simulink model "IEEE_BUS_68_Baseline"  (R2025a)
settings: Solver=ode23tb  StartTime=0.0  StopTime=150  FixedStep=Ts  MaxStep=0.0001  RelTol=1e-3
PreLoadFcn:
  | PSSMODEL=1;
  | LPSS=0;
  | WAPSS=0;
  | WAPSS2=0;
  | Ts=50e-5;
InitFcn:
  | PSSMODEL=1;
  | LPSS=0;
  | WAPSS=0;
  | WAPSS2=0;
  | Ts=50e-5;
  | 
  | % Required data to 68 Bus benchmark
  | % clear
  | % clc
  | % Definition for the columns
  | % system base =100 MVA
  | 
  | %% Line data Format (line)
  | % All values are given on the same system base MVA
  | % 1: From bus
  | % 2: To bus
  | % 3: Resistance (pu)
  | % 4: Reactance  (pu)
  | % 5: Charge     (pu)
  | % 6: Transformer Tap Amplitute
  | % 7: base MVA
  | % 8: Nomonal Voltage (KV)
  | 
  | %1   2    3        4       5       6        7      8
  | line=[...
  | 1	54	0	     0.0181	  0	      1.025     100    13.8
  | 2	58	0	     0.025	  0	      1.070     100    13.8
  | 3	62	0	     0.02	  0	      1.070     100    13.8
  | 4	19	0.0007	 0.0142	  0	      1.070     100    13.8
  | 5	20	0.0009	 0.018	  0	      1.009     100    13.8
  | 6	22	0	     0.0143	  0	      1.025     100    13.8
  | 7	23	0.0005	 0.0272	  0	      0         100    13.8
  | 8	25	0.0006	 0.0232	  0	      1.025     100    13.8
  | 9	29	0.0008	 0.0156   0	      1.025     100    13.8
  | 10	31	0	     0.026	  0	      1.04      100    13.8
  | 11	32	0	     0.013	  0	      1.04      100    13.8
  | 12	36	0	     0.0075	  0	      1.04      100    13.8
  | 13	17	0	     0.0033	  0	      1.04      100    13.8
  | 14	41	0	     0.0015	  0	      1         100    13.8
  | 15	42	0	     0.0015	  0	      1         100    13.8
  | 16	18	0	     0.003	  0	      1         100    13.8
  | 17	36	0.0005	 0.0045	  0.32	  0         100    138
  | 17	43	0.0005	 0.0276	  0	      0         100    138
  | 18	42	0.004	 0.06	  2.25    0         100    138
  | 18	49	0.0076	 0.1141	  1.16    0	        100    138
  | 18	50	0.0012	 0.0288	  2.06	  0         100    138
  | 20	19	0.0007	 0.0138	  0       1.06	    100    138
  | 19	68	0.0016	 0.0195	  0.304	  0         100    138
  | 21	22	0.0008	 0.014	  0.2565  0	        100    138
  | 21	68	0.0008	 0.0135	  0.2548  0	        100    138
  | 22	23	0.0006	 0.0096	  0.1846  0	        100    138
  | 23	24	0.0022	 0.035	  0.361	  0         100    138
  | 24	68	0.0003	 0.0059	  0.068	  0         100    138
  | 25	26	0.0032	 0.0323	  0.531	  0         100    138
  | 25	54	0.007	 0.0086	  0.146	  0         100    138
  | 26	27	0.0014	 0.0147	  0.2396  0	        100    138
  | 26	28	0.0043	 0.0474	  0.7802  0	        100    138
  | 26	29	0.0057	 0.0625	  1.029	  0         100    138
  | 27	37	0.0013	 0.0173	  0.3216  0	        100    138
  | 27	53	0.032	 0.32	  0.41	  0         100    138
  | 29	28	0.0014	 0.0151	  0.249	  0         100    138
  | 30	31	0.0013	 0.0187	  0.333	  0         100    138
  | 30	32	0.0024	 0.0288	  0.488	  0         100    138
  | 30	53	0.0008	 0.0074	  0.48	  0         100    138
  | 30	61	0.00095	 0.00915  0.58	  0         100    138
  | 31	38	0.0011	 0.0147	  0.247	  0         100    138
  | 31	53	0.0016	 0.0163	  0.25	  0         100    138
  | 32	33	0.0008	 0.0099	  0.168	  0         100    138
  | 33	34	0.0011	 0.0157	  0.202	  0         100    138
  | 33	38	0.0036	 0.0444	  0.693	  0         100    138
  | 34	35	0.0001	 0.0074	  0	      0.946     100    138
  | 34	36	0.0033	 0.0111	  1.45	  0         100    138
  | 35	45	0.0007	 0.0175	  1.39	  0         100    138
  | 36	61	0.0011	 0.0098	  0.68	  0         100    138
  | 37	52	0.0007	 0.0082	  0.1319  0	        100    138
  | 37	68	0.0007	 0.0089	  0.1342  0	        100    138
  | 38	46	0.0022	 0.0284	  0.43	  0         100    138
  | 39	44	0	     0.0411	  0	      0         100    138
  | 39	45	0	     0.0839	  0	      0         100    138
  | 40	41	0.006	 0.084	  3.15	  0         100    138
  | 40	48	0.002	 0.022	  1.28	  0         100    138
  | 41	42	0.004	 0.06	  2.25	  0         100    138
  | 43	44	0.0001	 0.0011	  0	      0         100    138
  | 44	45	0.0025	 0.073	  0	      0         100    138
  | 45	51	0.0004	 0.0105	  0.72	  0         100    138
  | 46	49	0.0018	 0.0274	  0.27	  0         100    138
  | 47	48	0.00125	 0.0134	  0.8	  0         100    138
  | 47	53	0.0013	 0.0188	  1.31	  0         100    138
  | 50	51	0.0009	 0.0221	  1.62	  0         100    138
  | 52	55	0.0011	 0.0133	  0.2138  0	        100    138
  | 53	54	0.0035	 0.0411	  0.6987  0	        100    138
  | 54	55	0.0013	 0.0151	  0.2572  0	        100    138
  | 55	56	0.0013	 0.0213	  0.2214  0	        100    138
  | 56	57	0.0008	 0.0128	  0.1342  0	        100    138
  | 56	66	0.0008	 0.0129	  0.1382  0	        100    138
  | 57	58	0.0002	 0.0026	  0.0434  0	        100    138
  | 57	60	0.0008	 0.0112	  0.1476  0	        100    138
  | 58	59	0.0006	 0.0092	  0.113	  0         100    138
  | 58	63	0.0007	 0.0082	  0.1389  0	        100    138
  | 59	60	0.0004	 0.0046	  0.078	  0         100    138
  | 60	61	0.0023	 0.0363	  0.3804  0	        100    138
  | 62	63	0.0004	 0.0043	  0.0729  0	        100    138
  | 62	65	0.0004	 0.0043	  0.0729  0	        100    138
  | 63	64	0.0016	 0.0435	  0	      1.06      100    138
  | 65	64	0.0016	 0.0435	  0	      1.06      100    138
  | 65	66	0.0009	 0.0101	  0.1723  0 	    100    138
  | 66	67	0.0018	 0.0217	  0.366	  0         100    138
  | 67	68	0.0009	 0.0094   0.171   0         100   138 ];
  | 
  | 
  | 
  | %% Power System Stabilizer Format (MB)
  | % Applied power system stabilizer is MBPSS with simplified settings
  | % Note: All machines use MBPSS with same configuration
  | % 1: Global gain (G)
  | % 2: Frequency of low frequency band (FL) Hz
  | % 3: Gain of low frequency band (KL)
  | % 4: Frequency of intermediate frequency band (FI) Hz
  | % 5: Gain of intermediate frequency band (KI)
  | % 6: Frequency of high frequency band (FH) Hz
  | % 7: Gain of high frequency band (KH)
  | %   1    2  3     4   5      6  7
  | MB=[1   0.2 30   1.25 40    12 160];
  | 
  | %% Excitation System format (AVR_Data)
  | % All machines use IEEE type 1 synchronous machine voltage regulator combined to an exciter
  | % 1. Low pass filter time constant (Tr) sec
  | % 2. Regulator gain (Ka)
  | % 3. regulator time constant (Ta) sec
  | % 4. Lead-lag compensator time constant (Tb) sec
  | % 5. Lead-lag compensator time constant (Tc) sec
  | % 6. Terminal voltage (pu)
  | % 7. Lower limit for regulator output (Emin)
  | % 8. Upper limit for regulator output (Emax)
  | %     1    2      3      4     5     6       7    8
  |   AVR_Data=[...
  |     0.01  200    0.015   10    1    1.03    -5    5
  |     0.01  200    0.015   10    1    1.03    -5    5
  |     0.01  200    0.015   10    1    1.03    -5    5
  |     0.01  200    0.015   10    1    1.03    -5    5
  |     0.01  200    0.015   10    1    1.03    -5    5
  |     0.01  200    0.015   10    1    1.03    -5    5
  |     0.01  200    0.015   10    1    1.03    -5    5
  |     0.01  200    0.015   10    1    1.03    -5    5
  |     0.01  200    0.015   10    1    1.03    -5    5
  |     0.01  200    0.015   10    1    1.03    -5    5
  |     0.01  200    0.015   10    1    1.03    -5    5
  |     0.01  200    0.015   10    1    1.03    -5    5
  |     0.01  200    0.015   10    1    1.03    -5    5
  |     0.01  200    0.015   10    1    1.03    -5    5
  |     0.01  200    0.015   10    1    1.03    -5    5
  |     0.01  200    0.015   10    1    1.03    -5    5];
  | 
  | C0=829.7e-9;
  | L0=3.220e-3;
  | R0=1;
  | Ns=120*60/(2); %Nominal speed of synchronous machines
  | s=10;
  | 
  | %% Machine Data Format (mac_con)
  | % 1.  Machine Number
  | % 2.  Bus Number
  | % 3.  Base MVA
  | % 4.  Leakage Reactance x_l(pu)
  | % 5.  Resistance r_a(pu)
  | % 6.  d-axis sychronous reactance x_d(pu)
  | % 7.  d-axis transient reactance x'_d(pu)
  | % 8.  d-axis subtransient reactance x"_d(pu)
  | % 9.  d-axis open-circuit time constant T'_do(sec),
  | % 10. d-axis open-circuit subtransient time constant T"_do(sec)
  | % 11. q-axis sychronous reactance x_q(pu)
  | % 12. q-axis transient reactance x'_q(pu)
  | % 13. q-axis subtransient reactance x"_q(pu)
  | % 14. q-axis open-circuit time constant T'_qo(sec)
  | % 15. q-axis open circuit subtransient time constant % T"_qo(sec)
  | % 16. inertia constant H(sec)
  | % 17. damping coefficient d_o(pu)
  | % 18. dampling coefficient d_1(pu)
  | % 19. bus number
  | % Note: all the following machines use sub-transient model
  | % 1  2     3      4      5     6     7    8      9    10    11    12    13    14    15    16    17    18  19
  | mac_con = [ 01 01 100 0.0125 0.0 0.1 0.031 0.025 10.2 0.05 0.069 0.0416667 0.025 1.5 0.035 42. 0 0 01 0 0; 02 02 100 0.035 0.0 0.295 0.0697 0.05 6.56 0.05 0.282 0.0933333 0.05 1.5 0.035 30.2 0 0 02 0 0; 03 03 100 0.0304 0.0 0.2495 0.0531 0.045 5.7 0.05 0.237 0.0714286 0.045 1.5 0.035 35.8 0 0 03 0 0; 04 04 100 0.0295 0.0 0.262 0.0436 0.035 5.69 0.05 0.258 0.0585714 0.035 1.5 0.035 28.6 0 0 04 0 0; 05 05 100 0.027 0.0 0.33 0.066 0.05 5.4 0.05 0.31 0.0883333 0.05 0.44 0.035 26. 0 0 05 0 0; 06 06 100 0.0224 0.0 0.254 0.05 0.04 7.3 0.05 0.241 0.0675000 0.04 0.4 0.035 34.8 0 0 06 0 0; 07 07 100 0.0322 0.0 0.295 0.049 0.04 5.66 0.05 0.292 0.0666667 0.04 1.5 0.035 26.4 0 0 07 0 0; 08 08 100 0.028 0.0 0.29 0.057 0.045 6.7 0.05 0.280 0.0766667 0.045 0.41 0.035 24.3 0 0 08 0 0; 09 09 100 0.0298 0.0 0.2106 0.057 0.045 4.79 0.05 0.205 0.0766667 0.045 1.96 0.035 34.5 0 0 09 0 0; 10 10 100 0.0199 0.0 0.169 0.0457 0.04 9.37 0.05 0.115 0.0615385 0.04 1.5 0.035 31.0 0 0 10 0 0; 11 11 100 0.0103 0.0 0.128 0.018 0.012 4.1 0.05 0.123 0.0241176 0.012 1.5 0.035 28.2 0 0 11 0 0; 12 12 100 0.022 0.0 0.101 0.031 0.025 7.4 0.05 0.095 0.0420000 0.025 1.5 0.035 92.3 0 0 12 0 0; 13 13 200 0.0030 0.0 0.0296 0.0055 0.004 5.9 0.05 0.0286 0.0074000 0.004 1.5 0.035 248.0 0 0 13 0 0; 14 14 100 0.0017 0.0 0.018 0.00285 0.0023 4.1 0.05 0.0173 0.0037931 0.0023 1.5 0.035 300.0 0 0 14 0 0; 15 15 100 0.0017 0.0 0.018 0.00285 0.0023 4.1 0.05 0.0173 0.0037931 0.0023 1.5 0.035 300.0 0 0 15 0 0; 16 16 200 0.0041 0.0 0.0356 0.0071 0.0055 7.8 0.05 0.0334 0.0095000 0.0055 1.5 0.035 225.0 0 0 16 0 0; ] ;
  | 
  | p0=[250/200 545/200 650/200 632/200 505/200 700/200 560/200 540/200 800/200 500/200 1000/200 1350/200 3591/6000 1785/3000 1000/3000 3379.57/6000];%'./1000;%Active Power Generation of PV units
  | Pn(1:16,1)=1; % Nominal Power
  | % PSSModel=1;%1:No pSS //1:MB
  | %% Bus data (Bus)
  | % 1. Bus number
  | % 2. Nominal phase-phase voltage
  | %    1    2
  | Bus = [ ...
  | 1	13.8
  | 2	13.8
  | 3	13.8
  | 4	13.8
  | 5	13.8
  | 6	13.8
  | 7	13.8
  | 8	13.8
  | 9	13.8
  | 10	13.8
  | 11	13.8
  | 12	13.8
  | 13	13.8
  | 14	13.8
  | 15	13.8
  | 16	13.8
  | 17	138
  | 18	138
  | 19	138
  | 20	138
  | 21	138
  | 22	138
  | 23	138
  | 24	138
  | 25	138
  | 26	138
  | 27	138
  | 28	138
  | 29	138
  | 30	138
  | 31	138
  | 32	138
  | 33	138
  | 34	138
  | 35	138
  | 36	138
  | 37	138
  | 38	138
  | 39	138
  | 40	138
  | 41	138
  | 42	138
  | 43	138
  | 44	138
  | 45	138
  | 46	138
  | 47	138
  | 48	138
  | 49	138
  | 50	138
  | 51	138
  | 52	138
  | 53	138
  | 54	138
  | 55	138
  | 56	138
  | 57	138
  | 58	138
  | 59	138
  | 60	138
  | 61	138
  | 62	138
  | 63	138
  | 64	138
  | 65	138
  | 66	138
  | 67	138
  | 68	138];
  | 
  |    zbase=(line(:,8).^2)./line(:,7);
  |    line(:,3)=line(:,3).*zbase;
  |    line(:,4)=line(:,4).*zbase/(120*pi);
  |    line(:,5)=line(:,5)./zbase/(120*pi);
  | 
  | %PSSMODEL=1;
undefined symbols (not defined in the file or in its folder): D1, Delta
libraries: spsRMSLib x73, spsThreePhaseVIMeasurementLib x69, spsLoadFlowBusLib x69, spsThreePhasePISectionLineLib x64, spsThreePhaseParallelRLCLoadLib x35, spsGenericPowerSystemStabilizerLib x32, spsThreePhaseSeriesRLCLoadLib x21, spsThreePhaseTransformerTwoWindingsLib x21, spsSynchronousMachinepuStandardLib x19, spsExcitationSystemLib x16, spsMultiBandPowerSystemStabilizerLib x16, spsSteamTurbineandGovernorLib x16
(part 1 of 7)
settings Model: Creator=rubai  LastModifiedBy=vmoudgil
settings SolverCC: AllowMultiTaskInputOutput=on  AlgebraicLoopSolver=TrustRegion  AutoInsertRateTranBlk=on
settings DebuggingCC: UnconnectedInputMsg=warning  UnconnectedOutputMsg=warning  UnconnectedLineMsg=warning
settings ModelReferenceCC: EnableRefExpFcnMdlSchedulingChecks=on
settings RTWCC: GPUComputeCapability=3.5

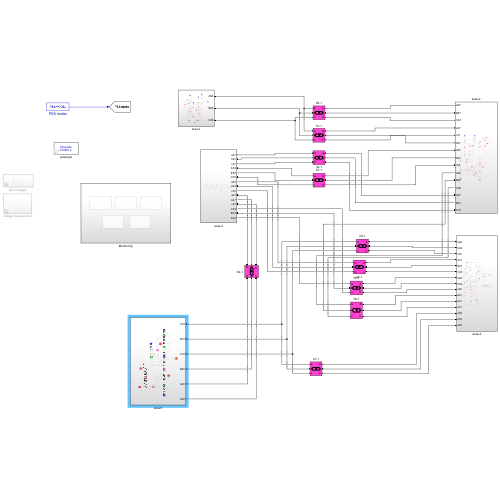
[thumbnail: Simulink's stored preview of the top-level diagram]
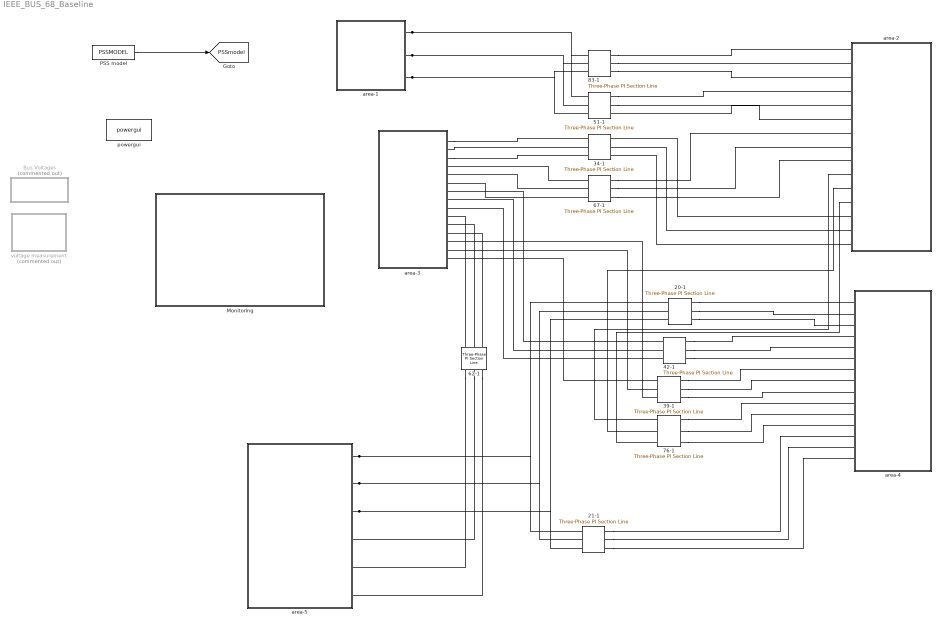
== system IEEE_BUS_68_Baseline ==
  20-1 : spsThreePhasePISectionLineLib/Three-Phase PI Section Line  LConnTagsString=a|b|c  RConnTagsString=A|B|C  Length=1  Frequency=60  Resistances=[line(20,3) 3*line(20,3)]  Inductances=[line(20,4) 3*line(20,4)]  Capacitances=[line(20,5) line(20,5)/3]
  21-1 : spsThreePhasePISectionLineLib/Three-Phase PI Section Line  LConnTagsString=a|b|c  RConnTagsString=A|B|C  Length=1  Frequency=60  Resistances=[line(21,3) 3*line(21,3)]  Inductances=[line(21,4) 3*line(21,4)]  Capacitances=[line(21,5) line(21,5)/3]
  34-1 : spsThreePhasePISectionLineLib/Three-Phase PI Section Line  LConnTagsString=a|b|c  RConnTagsString=A|B|C  Length=1  Frequency=60  Resistances=[line(34,3) 3*line(34,3)]  Inductances=[line(34,4) 3*line(34,4)]  Capacitances=[line(34,5) line(34,5)/3]
  39-1 : spsThreePhasePISectionLineLib/Three-Phase PI Section Line  LConnTagsString=a|b|c  RConnTagsString=A|B|C  Length=1  Frequency=60  Resistances=[line(39,3) 3*line(39,3)]  Inductances=[line(39,4) 3*line(39,4)]  Capacitances=[line(39,5) line(39,5)/3]
  42-1 : spsThreePhasePISectionLineLib/Three-Phase PI Section Line  LConnTagsString=a|b|c  RConnTagsString=A|B|C  Length=1  Frequency=60  Resistances=[line(42,3) 3*line(42,3)]  Inductances=[line(42,4) 3*line(42,4)]  Capacitances=[line(42,5) line(42,5)/3]
  51-1 : spsThreePhasePISectionLineLib/Three-Phase PI Section Line  LConnTagsString=a|b|c  RConnTagsString=A|B|C  Length=1  Frequency=60  Resistances=[line(51,3) 3*line(51,3)]  Inductances=[line(51,4) 3*line(51,4)]  Capacitances=[line(51,5) line(51,5)/3]
  62-1 : spsThreePhasePISectionLineLib/Three-Phase PI Section Line  LConnTagsString=a|b|c  RConnTagsString=A|B|C  Length=1  Frequency=60  Resistances=[line(62,3) 3*line(62,3)]  Inductances=[line(62,4) 3*line(62,4)]  Capacitances=[line(62,5) line(62,5)/3]
  67-1 : spsThreePhasePISectionLineLib/Three-Phase PI Section Line  LConnTagsString=a|b|c  RConnTagsString=A|B|C  Length=1  Frequency=60  Resistances=[line(67,3) 3*line(67,3)]  Inductances=[line(67,4) 3*line(67,4)]  Capacitances="[line(67,5)  line(67,5)/3]"
  76-1 : spsThreePhasePISectionLineLib/Three-Phase PI Section Line  LConnTagsString=a|b|c  RConnTagsString=A|B|C  Length=1  Frequency=60  Resistances=[line(76,3) 3*line(76,3)]  Inductances=[line(76,4) 3*line(76,4)]  Capacitances=[line(76,5) line(76,5)/3]
  83-1 : spsThreePhasePISectionLineLib/Three-Phase PI Section Line  LConnTagsString=a|b|c  RConnTagsString=A|B|C  Length=1  Frequency=60  Resistances=[line(83,3) 3*line(83,3)]  Inductances=[line(83,4) 3*line(83,4)]  Capacitances=[line(83,5) line(83,5)/3]
  "Bus Voltages " : Subsystem  Commented=on
  Monitoring : Subsystem
  PSS model : Constant  Value=PSSMODEL
  area-1 : Subsystem
  area-2 : Subsystem
  area-3 : Subsystem
  area-4 : Subsystem
  area-5 : Subsystem
  powergui : sps_lib/powergui  Priority=1  SimulationMode=Discrete  SampleTime=Ts  frequency=60  Iterations=1000  frequencyindice=60  Pbase=100e6  ErrMax=1e-4  UnitsV=kV  UnitsW=MW  buscounter=0  FunctionMessages=off  echomessages=off  EnableUseOfTLC=off  CurrentSourceSwitches=off  DisableSnubberDevices=off  DisableRonSwitches=off  DisableVfSwitches=off  DisplayEquations=off  AutomaticDiscreteSolvers=on  SolverType=Tustin/Backward Euler (TBE)  Interpol=off  ExternalGateDelay=off  methode=off  Ts=100  x0status=blocks  SPID=on  SwTol=0  HookPort=off  NonlinearTolerance=1e-4  nMaxIteration=100  ContinueOnMaxIteration=off  RestoreLinks=warning  ResistiveCurrentMeasurement=off  Frange=[0:2:500]  Ylog=off  Xlog=on  ShowGrid=off  save=off  variable=ZData  structure=0  ZoomFFT=off  StartTime=0.0  cycles=1  DisplayStyle=1  fundamental=60  FreqAxis=off  MaxFrequency=1000  frequencyindicesteady=1  RmsSteady=1  display=off
  "voltage measurement " : Subsystem  Commented=on
  tag scope: PSSmodel=global
  wires:
  PSS model/1 -> [PSSmodel]
  connections:
  area-5/RConn3 -- 21-1/RConn3 -- 20-1/RConn3
  area-1/RConn1 -- 51-1/RConn1 -- 83-1/RConn1
  area-1/RConn2 -- 51-1/RConn2 -- 83-1/RConn2
  area-5/RConn1 -- 21-1/RConn1 -- 20-1/RConn1
  area-1/RConn3 -- 51-1/RConn3 -- 83-1/RConn3
  area-5/RConn2 -- 21-1/RConn2 -- 20-1/RConn2
  67-1/LConn1 -- area-2/RConn7
  42-1/RConn3 -- area-4/RConn6
  51-1/LConn1 -- area-2/RConn4
  76-1/RConn2 -- area-2/RConn11
  20-1/LConn2 -- area-4/RConn2
  76-1/RConn3 -- area-2/RConn12
  62-1/LConn1 -- area-3/RConn10
  21-1/LConn2 -- area-4/RConn14
  42-1/RConn2 -- area-4/RConn5
  83-1/LConn3 -- area-2/RConn3
  area-3/RConn1 -- 34-1/LConn1
  42-1/LConn1 -- area-3/RConn7
  area-3/RConn3 -- 34-1/LConn3
  42-1/RConn1 -- area-4/RConn4
  39-1/RConn3 -- area-3/RConn13
  62-1/LConn3 -- area-3/RConn12
  62-1/RConn1 -- area-5/RConn5
  76-1/LConn1 -- area-4/RConn10
  39-1/RConn1 -- area-3/RConn15
  62-1/LConn2 -- area-3/RConn11
  83-1/LConn1 -- area-2/RConn1
  21-1/LConn3 -- area-4/RConn15
  20-1/LConn1 -- area-4/RConn1
  area-2/RConn14 -- 34-1/RConn2
  62-1/RConn3 -- area-5/RConn6
  62-1/RConn2 -- area-5/RConn4
  76-1/LConn3 -- area-4/RConn12
  area-2/RConn15 -- 34-1/RConn3
  67-1/RConn3 -- area-3/RConn6
  51-1/LConn2 -- area-2/RConn6
  67-1/LConn2 -- area-2/RConn8
  83-1/LConn2 -- area-2/RConn2
  67-1/LConn3 -- area-2/RConn9
  76-1/RConn1 -- area-2/RConn10
  39-1/LConn3 -- area-4/RConn9
  39-1/LConn1 -- area-4/RConn7
  39-1/LConn2 -- area-4/RConn8
  42-1/LConn3 -- area-3/RConn9
  39-1/RConn2 -- area-3/RConn14
  20-1/LConn3 -- area-4/RConn3
  67-1/RConn2 -- area-3/RConn5
  area-3/RConn2 -- 34-1/LConn2
  67-1/RConn1 -- area-3/RConn4
  42-1/LConn2 -- area-3/RConn8
  area-2/RConn5 -- 51-1/LConn3
  76-1/LConn2 -- area-4/RConn11
  21-1/LConn1 -- area-4/RConn13
  area-2/RConn13 -- 34-1/RConn1

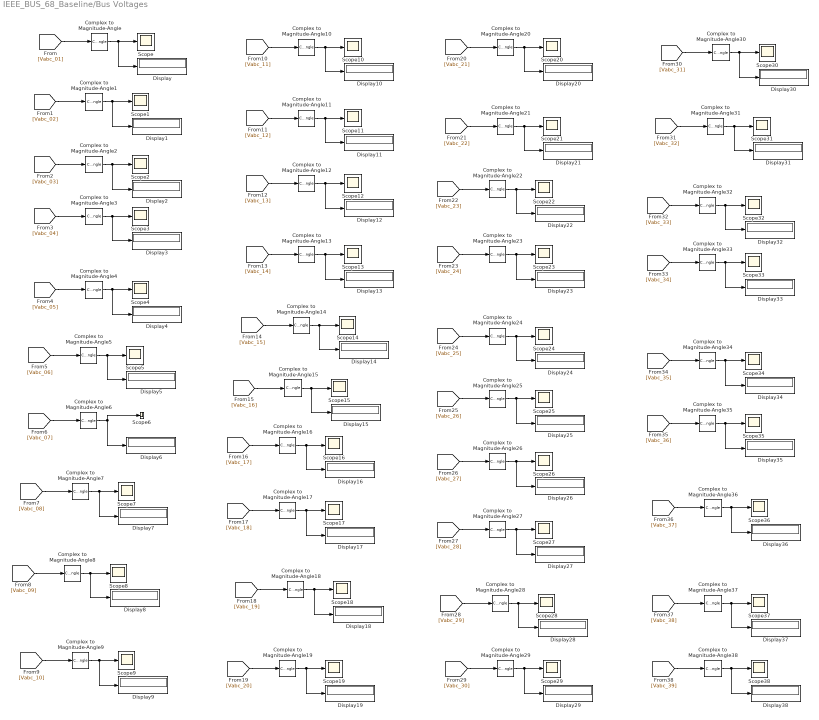
== system IEEE_BUS_68_Baseline/Bus Voltages  ==
  Complex to Magnitude-Angle{,1..38} (39 alike) : ComplexToMagnitudeAngle  Output=Magnitude
  Display{,1..38} (39 alike) : Display
  Scope{,1..38} (39 alike) : Scope
      Scope10 settings: DataLoggingVariableName=ScopeData10
      Scope11 settings: DataLoggingVariableName=ScopeData11
      Scope12 settings: DataLoggingVariableName=ScopeData12
      Scope13 settings: DataLoggingVariableName=ScopeData13
      Scope14 settings: DataLoggingVariableName=ScopeData14
      Scope15 settings: DataLoggingVariableName=ScopeData15
      Scope16 settings: DataLoggingVariableName=ScopeData16
      Scope17 settings: DataLoggingVariableName=ScopeData17
      Scope18 settings: DataLoggingVariableName=ScopeData18
      Scope19 settings: DataLoggingVariableName=ScopeData19
      Scope2 settings: DataLoggingVariableName=ScopeData2
      Scope20 settings: DataLoggingVariableName=ScopeData20
      Scope21 settings: DataLoggingVariableName=ScopeData21
      Scope22 settings: DataLoggingVariableName=ScopeData22
      Scope23 settings: DataLoggingVariableName=ScopeData23
      Scope24 settings: DataLoggingVariableName=ScopeData24
      Scope25 settings: DataLoggingVariableName=ScopeData25
      Scope26 settings: DataLoggingVariableName=ScopeData26
      Scope27 settings: DataLoggingVariableName=ScopeData27
      Scope28 settings: DataLoggingVariableName=ScopeData28
      Scope29 settings: DataLoggingVariableName=ScopeData29
      Scope3 settings: DataLoggingVariableName=ScopeData3
      Scope30 settings: DataLoggingVariableName=ScopeData30
      Scope31 settings: DataLoggingVariableName=ScopeData31
      Scope32 settings: DataLoggingVariableName=ScopeData32
      Scope33 settings: DataLoggingVariableName=ScopeData33
      Scope34 settings: DataLoggingVariableName=ScopeData34
      Scope35 settings: DataLoggingVariableName=ScopeData35
      Scope36 settings: DataLoggingVariableName=ScopeData36
      Scope37 settings: DataLoggingVariableName=ScopeData37
      Scope38 settings: DataLoggingVariableName=ScopeData38
      Scope4 settings: DataLoggingVariableName=ScopeData4
      Scope5 settings: DataLoggingVariableName=ScopeData5
      Scope6 settings: DataLoggingVariableName=ScopeData6
      Scope7 settings: DataLoggingVariableName=ScopeData7
      Scope8 settings: DataLoggingVariableName=ScopeData8
      Scope9 settings: DataLoggingVariableName=ScopeData9
  wires:
  [Vabc_01] -> Complex to Magnitude-Angle/1
  Complex to Magnitude-Angle/1 -> Display/1, Scope/1
  [Vabc_02] -> Complex to Magnitude-Angle1/1
  Complex to Magnitude-Angle1/1 -> Display1/1, Scope1/1
  [Vabc_03] -> Complex to Magnitude-Angle2/1
  Complex to Magnitude-Angle2/1 -> Display2/1, Scope2/1
  [Vabc_04] -> Complex to Magnitude-Angle3/1
  Complex to Magnitude-Angle3/1 -> Display3/1, Scope3/1
  [Vabc_05] -> Complex to Magnitude-Angle4/1
  Complex to Magnitude-Angle4/1 -> Display4/1, Scope4/1
  [Vabc_06] -> Complex to Magnitude-Angle5/1
  Complex to Magnitude-Angle5/1 -> Display5/1, Scope5/1
  [Vabc_07] -> Complex to Magnitude-Angle6/1
  Complex to Magnitude-Angle6/1 -> Display6/1, Scope6/1
  [Vabc_08] -> Complex to Magnitude-Angle7/1
  Complex to Magnitude-Angle7/1 -> Display7/1, Scope7/1
  [Vabc_09] -> Complex to Magnitude-Angle8/1
  Complex to Magnitude-Angle8/1 -> Display8/1, Scope8/1
  [Vabc_10] -> Complex to Magnitude-Angle9/1
  Complex to Magnitude-Angle9/1 -> Display9/1, Scope9/1
  [Vabc_11] -> Complex to Magnitude-Angle10/1
  Complex to Magnitude-Angle10/1 -> Display10/1, Scope10/1
  [Vabc_12] -> Complex to Magnitude-Angle11/1
  Complex to Magnitude-Angle11/1 -> Display11/1, Scope11/1
  [Vabc_13] -> Complex to Magnitude-Angle12/1
  Complex to Magnitude-Angle12/1 -> Display12/1, Scope12/1
  [Vabc_14] -> Complex to Magnitude-Angle13/1
  Complex to Magnitude-Angle13/1 -> Display13/1, Scope13/1
  [Vabc_15] -> Complex to Magnitude-Angle14/1
  Complex to Magnitude-Angle14/1 -> Display14/1, Scope14/1
  Complex to Magnitude-Angle15/1 -> Scope15/1, Display15/1
  [Vabc_16] -> Complex to Magnitude-Angle15/1
  [Vabc_17] -> Complex to Magnitude-Angle16/1
  Complex to Magnitude-Angle16/1 -> Display16/1, Scope16/1
  Complex to Magnitude-Angle17/1 -> Scope17/1, Display17/1
  [Vabc_18] -> Complex to Magnitude-Angle17/1
  [Vabc_19] -> Complex to Magnitude-Angle18/1
  Complex to Magnitude-Angle18/1 -> Display18/1, Scope18/1
  Complex to Magnitude-Angle19/1 -> Scope19/1, Display19/1
  [Vabc_20] -> Complex to Magnitude-Angle19/1
  Complex to Magnitude-Angle20/1 -> Scope20/1, Display20/1
  [Vabc_21] -> Complex to Magnitude-Angle20/1
  [Vabc_22] -> Complex to Magnitude-Angle21/1
  Complex to Magnitude-Angle21/1 -> Display21/1, Scope21/1
  Complex to Magnitude-Angle22/1 -> Scope22/1, Display22/1
  [Vabc_23] -> Complex to Magnitude-Angle22/1
  [Vabc_24] -> Complex to Magnitude-Angle23/1
  Complex to Magnitude-Angle23/1 -> Display23/1, Scope23/1
  Complex to Magnitude-Angle24/1 -> Scope24/1, Display24/1
  [Vabc_25] -> Complex to Magnitude-Angle24/1
  [Vabc_26] -> Complex to Magnitude-Angle25/1
  Complex to Magnitude-Angle25/1 -> Display25/1, Scope25/1
  Complex to Magnitude-Angle26/1 -> Scope26/1, Display26/1
  [Vabc_27] -> Complex to Magnitude-Angle26/1
  [Vabc_28] -> Complex to Magnitude-Angle27/1
  Complex to Magnitude-Angle27/1 -> Display27/1, Scope27/1
  Complex to Magnitude-Angle28/1 -> Scope28/1, Display28/1
  [Vabc_29] -> Complex to Magnitude-Angle28/1
  [Vabc_30] -> Complex to Magnitude-Angle29/1
  Complex to Magnitude-Angle29/1 -> Display29/1, Scope29/1
  Complex to Magnitude-Angle30/1 -> Scope30/1, Display30/1
  [Vabc_31] -> Complex to Magnitude-Angle30/1
  [Vabc_32] -> Complex to Magnitude-Angle31/1
  Complex to Magnitude-Angle31/1 -> Display31/1, Scope31/1
  Complex to Magnitude-Angle32/1 -> Scope32/1, Display32/1
  [Vabc_33] -> Complex to Magnitude-Angle32/1
  [Vabc_34] -> Complex to Magnitude-Angle33/1
  Complex to Magnitude-Angle33/1 -> Display33/1, Scope33/1
  Complex to Magnitude-Angle34/1 -> Scope34/1, Display34/1
  [Vabc_35] -> Complex to Magnitude-Angle34/1
  [Vabc_36] -> Complex to Magnitude-Angle35/1
  Complex to Magnitude-Angle35/1 -> Display35/1, Scope35/1
  Complex to Magnitude-Angle36/1 -> Scope36/1, Display36/1
  [Vabc_37] -> Complex to Magnitude-Angle36/1
  [Vabc_38] -> Complex to Magnitude-Angle37/1
  Complex to Magnitude-Angle37/1 -> Display37/1, Scope37/1
  Complex to Magnitude-Angle38/1 -> Scope38/1, Display38/1
  [Vabc_39] -> Complex to Magnitude-Angle38/1

== system IEEE_BUS_68_Baseline/Monitoring ==
  area1 : Subsystem
  area2 : Subsystem
  area3 : Subsystem
  area4 : Subsystem
  area5 : Subsystem

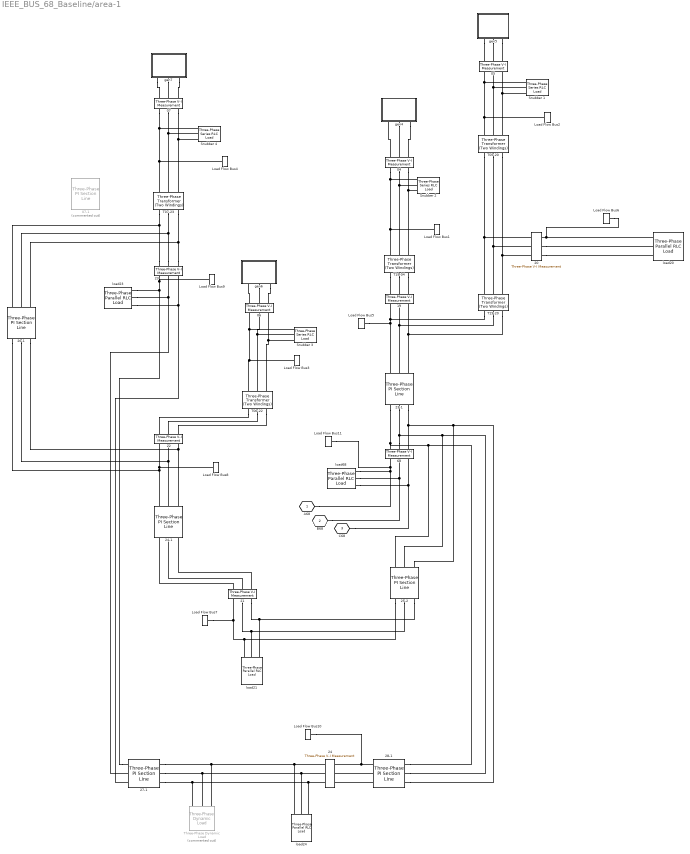
== system IEEE_BUS_68_Baseline/area-1 ==
  04 : spsThreePhaseVIMeasurementLib/Three-Phase V-I Measurement  VoltageMeasurement=phase-to-phase  SetLabelV=on  LabelV=Vabc_04  Vpu=off  VpuLL=on  CurrentMeasurement=no  SetLabelI=off  LabelI=Iabc  Ipu=off  Pbase=100e6  Vbase=13.8*1e3  OutputType=Complex  PhasorSimulation=off  PSBequivalent=0
  05 : spsThreePhaseVIMeasurementLib/Three-Phase V-I Measurement  VoltageMeasurement=phase-to-phase  SetLabelV=on  LabelV=Vabc_05  Vpu=off  VpuLL=on  CurrentMeasurement=no  SetLabelI=off  LabelI=Iabc  Ipu=off  Pbase=100e6  Vbase=13.8e3  OutputType=Complex  PhasorSimulation=off  PSBequivalent=0
  06 : spsThreePhaseVIMeasurementLib/Three-Phase V-I Measurement  VoltageMeasurement=phase-to-phase  SetLabelV=on  LabelV=Vabc_06  Vpu=off  VpuLL=on  CurrentMeasurement=no  SetLabelI=off  LabelI=Iabc  Ipu=off  Pbase=100e6  Vbase=13.8e3  OutputType=Complex  PhasorSimulation=off  PSBequivalent=0
  07 : spsThreePhaseVIMeasurementLib/Three-Phase V-I Measurement  VoltageMeasurement=phase-to-phase  SetLabelV=on  LabelV=Vabc_07  Vpu=off  VpuLL=on  CurrentMeasurement=no  SetLabelI=off  LabelI=Iabc  Ipu=off  Pbase=100e6  Vbase=13.8e3  OutputType=Complex  PhasorSimulation=off  PSBequivalent=0
  07-1 : spsThreePhasePISectionLineLib/Three-Phase PI Section Line  Commented=on  LConnTagsString=a|b|c  RConnTagsString=A|B|C  Length=1  Frequency=60  Resistances=[line(7,3) 3*line(7,3)]  Inductances=[line(7,4) 3*line(7,4)]  Capacitances=[line(28,5) line(28,5)/3]
  19 : spsThreePhaseVIMeasurementLib/Three-Phase V-I Measurement  VoltageMeasurement=phase-to-phase  SetLabelV=on  LabelV=Vabc_19  Vpu=off  VpuLL=on  CurrentMeasurement=no  SetLabelI=off  LabelI=Iabc  Ipu=off  Pbase=100e6  Vbase=Bus(19,2)*1e3  OutputType=Complex  PhasorSimulation=off  PSBequivalent=0
  20 : spsThreePhaseVIMeasurementLib/Three-Phase V-I Measurement  VoltageMeasurement=phase-to-phase  SetLabelV=on  LabelV=Vabc_20  Vpu=off  VpuLL=on  CurrentMeasurement=no  SetLabelI=off  LabelI=Iabc  Ipu=off  Pbase=100e6  Vbase=Bus(20,2)*1e3  OutputType=Complex  PhasorSimulation=off  PSBequivalent=0
  21 : spsThreePhaseVIMeasurementLib/Three-Phase V-I Measurement  VoltageMeasurement=phase-to-phase  SetLabelV=on  LabelV=Vabc_21  Vpu=off  VpuLL=on  CurrentMeasurement=no  SetLabelI=off  LabelI=Iabc  Ipu=off  Pbase=100e6  Vbase=Bus(21,2)*1e3  OutputType=Complex  PhasorSimulation=off  PSBequivalent=0
  22 : spsThreePhaseVIMeasurementLib/Three-Phase V-I Measurement  VoltageMeasurement=phase-to-phase  SetLabelV=on  LabelV=Vabc_22  Vpu=off  VpuLL=on  CurrentMeasurement=no  SetLabelI=off  LabelI=Iabc  Ipu=off  Pbase=100e6  Vbase=Bus(22,2)*1e3  OutputType=Complex  PhasorSimulation=off  PSBequivalent=0
  23 : spsThreePhaseVIMeasurementLib/Three-Phase V-I Measurement  VoltageMeasurement=phase-to-phase  SetLabelV=on  LabelV=Vabc_23  Vpu=off  VpuLL=on  CurrentMeasurement=no  SetLabelI=off  LabelI=Iabc  Ipu=off  Pbase=100e6  Vbase=Bus(23,2)*1e3  OutputType=Complex  PhasorSimulation=off  PSBequivalent=0
  23-1 : spsThreePhasePISectionLineLib/Three-Phase PI Section Line  LConnTagsString=a|b|c  RConnTagsString=A|B|C  Length=1  Frequency=60  Resistances="[line(23,3)  3*line(23,3)]"  Inductances=[line(23,4) 3*line(23,4)]  Capacitances=[line(23,5) line(23,5)/3]
  24 : spsThreePhaseVIMeasurementLib/Three-Phase V-I Measurement  VoltageMeasurement=phase-to-phase  SetLabelV=on  LabelV=Vabc_24  Vpu=off  VpuLL=on  CurrentMeasurement=no  SetLabelI=off  LabelI=Iabc  Ipu=off  Pbase=100e6  Vbase=Bus(24,2)*1e3  OutputType=Complex  PhasorSimulation=off  PSBequivalent=0
  24-1 : spsThreePhasePISectionLineLib/Three-Phase PI Section Line  LConnTagsString=a|b|c  RConnTagsString=A|B|C  Length=1  Frequency=60  Resistances=[line(24,3) 3*line(24,3)]  Inductances=[line(24,4) 3*line(24,4)]  Capacitances=[line(24,5) line(24,5)/3]
  25-2 : spsThreePhasePISectionLineLib/Three-Phase PI Section Line  LConnTagsString=a|b|c  RConnTagsString=A|B|C  Length=1  Frequency=60  Resistances=[line(25,3) 3*line(25,3)]  Inductances=[line(25,4) 3*line(25,4)]  Capacitances=[line(25,5) line(25,5)/3]
  26-1 : spsThreePhasePISectionLineLib/Three-Phase PI Section Line  LConnTagsString=a|b|c  RConnTagsString=A|B|C  Length=1  Frequency=60  Resistances=[line(26,3) 3*line(26,3)]  Inductances=[line(26,4) 3*line(26,4)]  Capacitances=[line(26,5) line(26,5)/3]
  27-1 : spsThreePhasePISectionLineLib/Three-Phase PI Section Line  LConnTagsString=a|b|c  RConnTagsString=A|B|C  Length=1  Frequency=60  Resistances=[line(27,3) 3*line(27,3)]  Inductances=[line(27,4) 3*line(27,4)]  Capacitances=[line(27,5) line(27,5)/3]
  28-1 : spsThreePhasePISectionLineLib/Three-Phase PI Section Line  LConnTagsString=a|b|c  RConnTagsString=A|B|C  Length=1  Frequency=60  Resistances=[line(28,3) 3*line(28,3)]  Inductances=[line(28,4) 3*line(28,4)]  Capacitances=[line(28,5) line(28,5)/3]
  68 : spsThreePhaseVIMeasurementLib/Three-Phase V-I Measurement  VoltageMeasurement=phase-to-phase  SetLabelV=on  LabelV=Vabc_68  Vpu=off  VpuLL=on  CurrentMeasurement=no  SetLabelI=off  LabelI=Iabc  Ipu=off  Pbase=100e6  Vbase=Bus(68,2)*1e3  OutputType=Complex  PhasorSimulation=off  PSBequivalent=0
  Load Flow Bus1 : spsLoadFlowBusLib/Load Flow Bus  LConnTagsString=a  Phases=single  Connectors=on one side  ID=BUS_04  Vbase=13.8e3  Vref=0.997  Vangle=0  VLF=0.997  VLFb=1  VLFc=1  angleLF=7.878  angleLFb=0  angleLFc=0
  Load Flow Bus10 : spsLoadFlowBusLib/Load Flow Bus  LConnTagsString=a  Phases=single  Connectors=on one side  ID=BUS_24  Vbase=138e3  Vref=1  Vangle=0  VLF=1.017  VLFb=1  VLFc=1  angleLF=27.85  angleLFb=0  angleLFc=0
  Load Flow Bus11 : spsLoadFlowBusLib/Load Flow Bus  LConnTagsString=a  Phases=single  Connectors=on one side  ID=BUS_68  Vbase=138e3  Vref=1  Vangle=0  VLF=1.009  VLFb=1  VLFc=1  angleLF=27.68  angleLFb=0  angleLFc=0
  Load Flow Bus2 : spsLoadFlowBusLib/Load Flow Bus  LConnTagsString=a  Phases=single  Connectors=on one side  ID=BUS_05  Vbase=13.8e3  Vref=1.011  Vangle=0  VLF=1.011  VLFb=1  VLFc=1  angleLF=3.855  angleLFb=0  angleLFc=0
  Load Flow Bus3 : spsLoadFlowBusLib/Load Flow Bus  LConnTagsString=a  Phases=single  Connectors=on one side  ID=BUS_06  Vbase=13.8e3  Vref=1.05  Vangle=0  VLF=1.05  VLFb=1  VLFc=1  angleLF=7.781  angleLFb=0  angleLFc=0
  Load Flow Bus4 : spsLoadFlowBusLib/Load Flow Bus  LConnTagsString=a  Phases=single  Connectors=on one side  ID=BUS_07  Vbase=13.8e3  Vref=1.063  Vangle=0  VLF=1.063  VLFb=1  VLFc=1  angleLF=8.754  angleLFb=0  angleLFc=0
  Load Flow Bus5 : spsLoadFlowBusLib/Load Flow Bus  LConnTagsString=a  Phases=single  Connectors=on one side  ID=BUS_19  Vbase=138e3  Vref=1  Vangle=0  VLF=0.9998  VLFb=1  VLFc=1  angleLF=32.72  angleLFb=0  angleLFc=0
  Load Flow Bus6 : spsLoadFlowBusLib/Load Flow Bus  LConnTagsString=a  Phases=single  Connectors=on one side  ID=BUS_20  Vbase=138e3  Vref=1  Vangle=0  VLF=0.9971  VLFb=1  VLFc=1  angleLF=31.31  angleLFb=0  angleLFc=0
  Load Flow Bus7 : spsLoadFlowBusLib/Load Flow Bus  LConnTagsString=a  Phases=single  Connectors=on one side  ID=BUS_21  Vbase=138e3  Vref=1  Vangle=0  VLF=1.014  VLFb=1  VLFc=1  angleLF=30.37  angleLFb=0  angleLFc=0
  Load Flow Bus8 : spsLoadFlowBusLib/Load Flow Bus  LConnTagsString=a  Phases=single  Connectors=on one side  ID=BUS_22  Vbase=138e3  Vref=1  Vangle=0  VLF=1.039  VLFb=1  VLFc=1  angleLF=35.14  angleLFb=0  angleLFc=0
  Load Flow Bus9 : spsLoadFlowBusLib/Load Flow Bus  LConnTagsString=a  Phases=single  Connectors=on one side  ID=BUS_23  Vbase=138e3  Vref=1  Vangle=0  VLF=1.039  VLFb=1  VLFc=1  angleLF=34.82  angleLFb=0  angleLFc=0
  Snubber {1..4} (4 alike) : spsThreePhaseSeriesRLCLoadLib/Three-Phase Series RLC Load  LConnTagsString=A|B|C  Configuration=Y (grounded)  NominalVoltage=13.8e3  Vabc=[1e3 1e3 1e3]  Vabcp=[1e3 1e3 1e3]  NominalFrequency=60  UnbalancedPower=off  ActivePower=1000000  InductivePower=0  CapacitivePower=10000000  Pabc=[10e3 9e3 11e3]  QLabc=[100 90 110]  QCabc=[100 90 110]  Pabcp=[10e3 9e3 11e3]  QLabcp=[100 90 110]  QCabcp=[100 90 110]  Measurements=None  LoadType=constant Z
  T05-20 : spsThreePhaseTransformerTwoWindingsLib/Three-Phase Transformer (Two Windings)  Winding1Connection=Delta (D1)  Winding2Connection=Yg  CoreType=Three single-phase transformers  SetSaturation=off  Hysteresis=off  DataFile='hysteresis'  SetInitialFlux=off  Measurements=None  UNITS=pu  NominalPower=[ 100e6 , 60 ]  Winding1=[ 13.8e3 , 0.0, 0 ]  Winding2=[ 138e3 , 0.00085, 0.0091]  Rm=500  Lm=500  L0=0.5  Saturation=[ 0,0 ; 0.0024,1.2 ; 1.0,1.52 ]  InitialFluxes=[ 0.8 , -0.8 , 0.7 ]  BreakLoop=off  DiscreteSolver=Trapezoidal robust  DataType=off  TransfoNumber=1
  T06-22 : spsThreePhaseTransformerTwoWindingsLib/Three-Phase Transformer (Two Windings)  Winding1Connection=Delta (D1)  Winding2Connection=Yg  CoreType=Three single-phase transformers  SetSaturation=off  Hysteresis=off  DataFile='hysteresis'  SetInitialFlux=off  Measurements=None  UNITS=pu  NominalPower=[ 100e6 , 60 ]  Winding1=[ 13.8e3 , 0.00 , 0 ]  Winding2=[ 138e3 , 0.000 , 0.0072 ]  Rm=500  Lm=500  L0=0.5  Saturation=[ 0,0 ; 0.0024,1.2 ; 1.0,1.52 ]  InitialFluxes=[ 0.8 , -0.8 , 0.7 ]  BreakLoop=off  DiscreteSolver=Trapezoidal robust  DataType=off  TransfoNumber=1
  T07-23 : spsThreePhaseTransformerTwoWindingsLib/Three-Phase Transformer (Two Windings)  Winding1Connection=Delta (D1)  Winding2Connection=Yg  CoreType=Three single-phase transformers  SetSaturation=off  Hysteresis=off  DataFile='hysteresis'  SetInitialFlux=off  Measurements=None  UNITS=pu  NominalPower=[ 100e6 , 60 ]  Winding1=[ 13.8e3 , 0.00035 , 0 ]  Winding2=[ 138e3 , 0.00035, 0.0138]  Rm=500  Lm=500  L0=0.5  Saturation=[ 0,0 ; 0.0024,1.2 ; 1.0,1.52 ]  InitialFluxes=[ 0.8 , -0.8 , 0.7 ]  BreakLoop=off  DiscreteSolver=Trapezoidal robust  DataType=off  TransfoNumber=1
  T19-04 : spsThreePhaseTransformerTwoWindingsLib/Three-Phase Transformer (Two Windings)  Winding1Connection=Delta (D1)  Winding2Connection=Yg  CoreType=Three single-phase transformers  SetSaturation=off  Hysteresis=off  DataFile='hysteresis'  SetInitialFlux=off  Measurements=None  UNITS=pu  NominalPower=[ 100e6 , 60 ]  Winding1=[ 13.8e3 , 0.00035 , 0 ]  Winding2=[ 138e3 , 0.000035, 0.0142]  Rm=500  Lm=500  L0=0.5  Saturation=[ 0,0 ; 0.0024,1.2 ; 1.0,1.52 ]  InitialFluxes=[ 0.8 , -0.8 , 0.7 ]  BreakLoop=off  DiscreteSolver=Trapezoidal robust  DataType=off  TransfoNumber=1
  T19-20 : spsThreePhaseTransformerTwoWindingsLib/Three-Phase Transformer (Two Windings)  Winding1Connection=Y  Winding2Connection=Y  CoreType=Three single-phase transformers  SetSaturation=off  Hysteresis=off  DataFile='hysteresis'  SetInitialFlux=off  Measurements=None  UNITS=pu  NominalPower=[ 100e6 , 60 ]  Winding1=[ 138e3 , 0.00035 , 0 ]  Winding2=[ 138e3 , 0.00035, 0.0138]  Rm=500  Lm=500  L0=0.5  Saturation=[ 0,0 ; 0.0024,1.2 ; 1.0,1.52 ]  InitialFluxes=[ 0.8 , -0.8 , 0.7 ]  BreakLoop=off  DiscreteSolver=Trapezoidal robust  DataType=off  TransfoNumber=1
  Three-Phase Dynamic Load : spsThreePhaseDynamicLoadLib/Three-Phase Dynamic Load  Commented=on  NominalVoltage=[138000 60 ]  ActiveReactivePowers=[309000000 -92000000]  PositiveSequence=[1.01116 21.5615]  ExternalControl=off  NpNq=[1.3 2]  TimeConstants=[0.1 0.1 0.1 0.1]  MinimumVoltage=0.5  Tfilter=0.01  LoadFlowParameters=[4,0,0,0,0]
      settings: LibrarySourceBlock=|
      | sps_lib/Passives/Three-Phase
      | Dynamic Load
  gen4 : Subsystem
  gen5 : Subsystem
  gen6 : Subsystem
  gen7 : Subsystem
  load20 : spsThreePhaseParallelRLCLoadLib/Three-Phase Parallel RLC Load  LConnTagsString=A|B|C  Configuration=Y (grounded)  NominalVoltage=(138000)*0.997057  Vabc=[1e3 1e3 1e3]  Vabcp=[1e3 1e3 1e3]  NominalFrequency=60  UnbalancedPower=off  ActivePower=680000000  InductivePower=103000000  CapacitivePower=0  Pabc=[10e3 9e3 11e3]  QLabc=[100 90 110]  QCabc=[100 90 110]  Pabcp=[10e3 9e3 11e3]  QLabcp=[100 90 110]  QCabcp=[100 90 110]  Measurements=None  LoadType=constant PQ
  load21 : spsThreePhaseParallelRLCLoadLib/Three-Phase Parallel RLC Load  LConnTagsString=A|B|C  Configuration=Y (grounded)  NominalVoltage=(138000)*1.0142  Vabc=[1e3 1e3 1e3]  Vabcp=[1e3 1e3 1e3]  NominalFrequency=60  UnbalancedPower=off  ActivePower=274000000  InductivePower=115000000  CapacitivePower=0  Pabc=[10e3 9e3 11e3]  QLabc=[100 90 110]  QCabc=[100 90 110]  Pabcp=[10e3 9e3 11e3]  QLabcp=[100 90 110]  QCabcp=[100 90 110]  Measurements=None  LoadType=constant PQ
  load23 : spsThreePhaseParallelRLCLoadLib/Three-Phase Parallel RLC Load  LConnTagsString=A|B|C  Configuration=Y (grounded)  NominalVoltage=(138000)*1.0394  Vabc=[1e3 1e3 1e3]  Vabcp=[1e3 1e3 1e3]  NominalFrequency=60  UnbalancedPower=off  ActivePower=248000000  InductivePower=85000000  CapacitivePower=0  Pabc=[10e3 9e3 11e3]  QLabc=[100 90 110]  QCabc=[100 90 110]  Pabcp=[10e3 9e3 11e3]  QLabcp=[100 90 110]  QCabcp=[100 90 110]  Measurements=None  LoadType=constant PQ
  load24 : spsThreePhaseParallelRLCLoadLib/Three-Phase Parallel RLC Load  LConnTagsString=A|B|C  Configuration=Y (grounded)  NominalVoltage=(138000)*1.01663  Vabc=[1e3 1e3 1e3]  Vabcp=[1e3 1e3 1e3]  NominalFrequency=60  UnbalancedPower=off  ActivePower=309000000  InductivePower=0  CapacitivePower=92000000  Pabc=[10e3 9e3 11e3]  QLabc=[100 90 110]  QCabc=[100 90 110]  Pabcp=[10e3 9e3 11e3]  QLabcp=[100 90 110]  QCabcp=[100 90 110]  Measurements=None  LoadType=constant PQ
  load68 : spsThreePhaseParallelRLCLoadLib/Three-Phase Parallel RLC Load  LConnTagsString=A|B|C  Configuration=Y (grounded)  NominalVoltage=(138000)*1.00862  Vabc=[1e3 1e3 1e3]  Vabcp=[1e3 1e3 1e3]  NominalFrequency=60  UnbalancedPower=off  ActivePower=329000000  InductivePower=32000000  CapacitivePower=0  Pabc=[10e3 9e3 11e3]  QLabc=[100 90 110]  QCabc=[100 90 110]  Pabcp=[10e3 9e3 11e3]  QLabcp=[100 90 110]  QCabcp=[100 90 110]  Measurements=None  LoadType=constant PQ
  A68 : PMIOPort  Tag=PMCPort  Side=Right
  B68 : PMIOPort  Tag=PMCPort  Port=2  Side=Right
  C68 : PMIOPort  Tag=PMCPort  Port=3  Side=Right
  connections:
  B68/RConn1 -- load68/LConn2 -- 68/LConn2
  27-1/LConn1 -- Load Flow Bus9/LConn1 -- 23/LConn1 -- load23/LConn1
  T19-20/LConn3 -- T05-20/RConn3 -- 20/RConn3
  20/RConn1 -- T05-20/RConn1 -- T19-20/LConn1
  24-1/RConn1 -- 26-1/RConn1 -- Load Flow Bus8/LConn1 -- 22/LConn1
  04/LConn2 -- T19-04/LConn2 -- Snubber 2/LConn2
  07/LConn1 -- Snubber 4/LConn1 -- Load Flow Bus4/LConn1 -- T07-23/LConn1
  07/LConn3 -- T07-23/LConn3 -- Snubber 4/LConn3
  load23/LConn2 -- 23/LConn2 -- 27-1/LConn2
  21/LConn3 -- load21/LConn3 -- 25-2/RConn3
  24-1/RConn3 -- 22/LConn3 -- 26-1/RConn3
  04/LConn1 -- Snubber 2/LConn1 -- Load Flow Bus1/LConn1 -- T19-04/LConn1
  A68/RConn1 -- load68/LConn1 -- 68/LConn1 -- Load Flow Bus11/LConn1
  04/RConn1 -- gen4/LConn1
  T19-20/LConn2 -- T05-20/RConn2 -- 20/RConn2
  23-1/RConn1 -- Load Flow Bus5/LConn1 -- T19-20/RConn1 -- 19/LConn1
  21/LConn2 -- load21/LConn2 -- 25-2/RConn2
  load23/LConn3 -- 23/LConn3 -- 27-1/LConn3
  T06-22/RConn3 -- 22/RConn3
  07/LConn2 -- Snubber 4/LConn2 -- T07-23/LConn2
  load21/LConn1 -- Load Flow Bus7/LConn1 -- 21/LConn1 -- 25-2/RConn1
  C68/RConn1 -- load68/LConn3 -- 68/LConn3
  T06-22/LConn1 -- Load Flow Bus3/LConn1 -- Snubber 3/LConn1 -- 06/LConn1
  T05-20/LConn1 -- Load Flow Bus2/LConn1 -- Snubber 1/LConn1 -- 05/LConn1
  T06-22/LConn3 -- 06/LConn3 -- Snubber 3/LConn3
  26-1/RConn2 -- 24-1/RConn2 -- 22/LConn2
  T06-22/LConn2 -- Snubber 3/LConn2 -- 06/LConn2
  04/LConn3 -- Snubber 2/LConn3 -- T19-04/LConn3
  T06-22/RConn2 -- 22/RConn2
  gen4/LConn2 -- 04/RConn2
  23-1/LConn1 -- 68/RConn1 -- 28-1/LConn1 -- 25-2/LConn1
  T19-04/RConn3 -- 19/RConn3
  68/RConn2 -- 23-1/LConn2 -- 28-1/LConn2 -- 25-2/LConn2
  T06-22/RConn1 -- 22/RConn1
  T19-04/RConn2 -- 19/RConn2
  28-1/LConn3 -- 68/RConn3 -- 23-1/LConn3 -- 25-2/LConn3
  gen4/LConn3 -- 04/RConn3
  19/LConn2 -- 23-1/RConn2 -- T19-20/RConn2
  T19-04/RConn1 -- 19/RConn1
  T05-20/LConn2 -- Snubber 1/LConn2 -- 05/LConn2
  T05-20/LConn3 -- Snubber 1/LConn3 -- 05/LConn3
  gen5/LConn1 -- 05/RConn1
  gen5/LConn2 -- 05/RConn2
  gen5/LConn3 -- 05/RConn3
  06/RConn1 -- gen6/LConn1
  gen6/LConn2 -- 06/RConn2
  gen6/LConn3 -- 06/RConn3
  gen7/LConn1 -- 07/RConn1
  gen7/LConn2 -- 07/RConn2
  gen7/LConn3 -- 07/RConn3
  19/LConn3 -- 23-1/RConn3 -- T19-20/RConn3
  23/RConn1 -- T07-23/RConn1 -- 26-1/LConn1
  23/RConn2 -- T07-23/RConn2 -- 26-1/LConn2
  23/RConn3 -- T07-23/RConn3 -- 26-1/LConn3
  21/RConn1 -- 24-1/LConn1
  21/RConn2 -- 24-1/LConn2
  21/RConn3 -- 24-1/LConn3
  28-1/RConn1 -- 24/LConn1 -- Load Flow Bus10/LConn1
  28-1/RConn2 -- 24/LConn2
  28-1/RConn3 -- 24/LConn3
  Load Flow Bus6/LConn1 -- load20/LConn1 -- 20/LConn1
  27-1/RConn1 -- load24/LConn1 -- 24/RConn1 -- Three-Phase Dynamic Load/LConn1
  24/RConn2 -- Three-Phase Dynamic Load/LConn2 -- 27-1/RConn2 -- load24/LConn2
  24/RConn3 -- Three-Phase Dynamic Load/LConn3 -- 27-1/RConn3 -- load24/LConn3
  20/LConn2 -- load20/LConn2
  20/LConn3 -- load20/LConn3
